simulink library "bushing_forces_lib"  (R2025a)
settings: Solver=VariableStepAuto  StartTime=0.0  StopTime=10.0  RelTol=1e-3
undefined symbols (not defined in the file): b1_radial_max, d_axial, d_axialX, d_axialY, d_axialZ, d_radial, d_tors, d_torsX, d_torsY, d_torsZ, f_axial_dam, f_axial_spr, f_axialX_dam, f_axialX_spr, f_axialY_dam, f_axialY_spr, f_axialZ_dam, f_axialZ_spr, f_radial_dam, f_radial_max, f_radial_spr, k1_radial_max, k_axial, k_axialX, k_axialY, k_axialZ, k_radial, k_tors, k_torsX, k_torsY, k_torsZ, Linear, m, m_spr, m_sprZ, m_torsY, m_torsZ, m_torX, q_spr, q_sprZ, Table, v_axial, v_axialX, v_axialY, v_axialZ, v_radial, w, w_torsY, w_torsZ, w_torX, x_axial, x_axialX, x_axialY, x_axialZ, x_radial, x_radial_max
libraries: nesl_utility x26, fl_lib x18, $bdroot x10
(part 2 of 2)

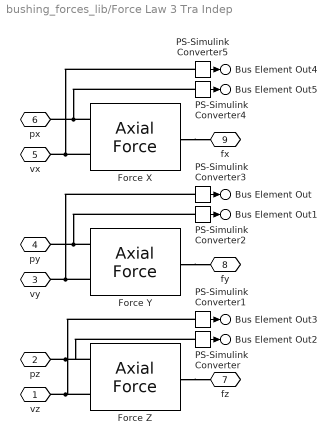
== system bushing_forces_lib/Force Law 3 Tra Indep ==
  Force X : $bdroot/Axial Force  popup_force_law_spr=Linear  k_axial=k_axialX  x_axial=x_axialX  f_axial_spr=f_axialX_spr  popup_force_law_dam=Linear  d_axial=d_axialX  v_axial=v_axialX  f_axial_dam=f_axialX_dam
  Force Y : $bdroot/Axial Force  popup_force_law_spr=Linear  k_axial=k_axialY  x_axial=x_axialY  f_axial_spr=f_axialY_spr  popup_force_law_dam=Linear  d_axial=d_axialY  v_axial=v_axialY  f_axial_dam=f_axialY_dam
  Force Z : $bdroot/Axial Force  popup_force_law_spr=Linear  k_axial=k_axialZ  x_axial=x_axialZ  f_axial_spr=f_axialZ_spr  popup_force_law_dam=Linear  d_axial=d_axialZ  v_axial=v_axialZ  f_axial_dam=f_axialZ_dam
  PS-Simulink Converter : nesl_utility/PS-Simulink Converter  PhysicalDomain=network_engine_domain  SubClassName=ps_output  LeftPortType=input  RightPortType=output  PseudoPeriodic=off  Frequencies=[]  VectorFormat=inherit  Unit=mm  AffineConversion=off
  PS-Simulink Converter1 : nesl_utility/PS-Simulink Converter  PhysicalDomain=network_engine_domain  SubClassName=ps_output  LeftPortType=input  RightPortType=output  PseudoPeriodic=off  Frequencies=[]  VectorFormat=inherit  Unit=m/s  AffineConversion=off
  PS-Simulink Converter2 : nesl_utility/PS-Simulink Converter  PhysicalDomain=network_engine_domain  SubClassName=ps_output  LeftPortType=input  RightPortType=output  PseudoPeriodic=off  Frequencies=[]  VectorFormat=inherit  Unit=mm  AffineConversion=off
  PS-Simulink Converter3 : nesl_utility/PS-Simulink Converter  PhysicalDomain=network_engine_domain  SubClassName=ps_output  LeftPortType=input  RightPortType=output  PseudoPeriodic=off  Frequencies=[]  VectorFormat=inherit  Unit=m/s  AffineConversion=off
  PS-Simulink Converter4 : nesl_utility/PS-Simulink Converter  PhysicalDomain=network_engine_domain  SubClassName=ps_output  LeftPortType=input  RightPortType=output  PseudoPeriodic=off  Frequencies=[]  VectorFormat=inherit  Unit=mm  AffineConversion=off
  PS-Simulink Converter5 : nesl_utility/PS-Simulink Converter  PhysicalDomain=network_engine_domain  SubClassName=ps_output  LeftPortType=input  RightPortType=output  PseudoPeriodic=off  Frequencies=[]  VectorFormat=inherit  Unit=m/s  AffineConversion=off
  vz : PMIOPort  Side=Right
  pz : PMIOPort  Port=2  Side=Right
  vy : PMIOPort  Port=3  Side=Right
  py : PMIOPort  Port=4  Side=Right
  vx : PMIOPort  Port=5  Side=Right
  px : PMIOPort  Port=6  Side=Right
  fz : PMIOPort  Port=7  Side=Left
  fy : PMIOPort  Port=8  Side=Left
  fx : PMIOPort  Port=9  Side=Left
  Bus Element Out : Outport  PortName=m  Element=vy
  Bus Element Out1 : Outport  PortName=m  Element=py
  Bus Element Out2 : Outport  PortName=m  Element=pz
  Bus Element Out3 : Outport  PortName=m  Element=vz
  Bus Element Out4 : Outport  PortName=m  Element=vx
  Bus Element Out5 : Outport  PortName=m  Element=px
  wires:
  PS-Simulink Converter1/1 -> Bus Element Out3/1
  PS-Simulink Converter/1 -> Bus Element Out2/1
  PS-Simulink Converter3/1 -> Bus Element Out/1
  PS-Simulink Converter2/1 -> Bus Element Out1/1
  PS-Simulink Converter4/1 -> Bus Element Out5/1
  PS-Simulink Converter5/1 -> Bus Element Out4/1
  connections:
  vz/RConn1 -- Force Z/LConn2 -- PS-Simulink Converter1/LConn1
  Force Z/RConn1 -- fz/RConn1
  pz/RConn1 -- Force Z/LConn1 -- PS-Simulink Converter/LConn1
  Force Y/RConn1 -- fy/RConn1
  Force X/RConn1 -- fx/RConn1
  PS-Simulink Converter2/LConn1 -- Force Y/LConn1 -- py/RConn1
  PS-Simulink Converter4/LConn1 -- Force X/LConn1 -- px/RConn1
  PS-Simulink Converter5/LConn1 -- Force X/LConn2 -- vx/RConn1
  PS-Simulink Converter3/LConn1 -- Force Y/LConn2 -- vy/RConn1

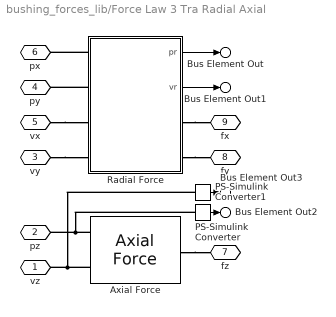
== system bushing_forces_lib/Force Law 3 Tra Radial Axial ==
  Axial Force : $bdroot/Axial Force  popup_force_law_spr=Linear  k_axial=k_axial  x_axial=x_axial  f_axial_spr=f_axial_spr  popup_force_law_dam=Linear  d_axial=d_axial  v_axial=v_axial  f_axial_dam=f_axial_dam
  PS-Simulink Converter : nesl_utility/PS-Simulink Converter  PhysicalDomain=network_engine_domain  SubClassName=ps_output  LeftPortType=input  RightPortType=output  PseudoPeriodic=off  Frequencies=[]  VectorFormat=inherit  Unit=mm  AffineConversion=off
  PS-Simulink Converter1 : nesl_utility/PS-Simulink Converter  PhysicalDomain=network_engine_domain  SubClassName=ps_output  LeftPortType=input  RightPortType=output  PseudoPeriodic=off  Frequencies=[]  VectorFormat=inherit  Unit=m/s  AffineConversion=off
  Radial Force : Subsystem  mask(Radial Compliance){popup_force_law_spr=Linear, k_radial=k_radial, f_radial_spr=f_radial_spr, x_radial=x_radial, k1_radial_max=k1_radial_max, b1_radial_max=b1_radial_max, x_radial_max=x_radial_max, f_radial_max=f_radial_max, popup_force_law_dam=Linear, d_radial=d_radial, v_radial=v_radial, f_radial_dam=f_radial_dam}
      mask prompts: popup_force_law_spr "Spring Force Law"; k_radial "Spring Coefficient (N/mm)"; f_radial_spr "Spring Force [min max] (N)"; x_radial "Spring Deflection [min max] (mm)"; k1_radial_max "Maxwell k1"; b1_radial_max "Maxwell b1"; x_radial_max "Maxwell Displacement [min max] (mm)"; f_radial_max "Maxwell Force [min max] (N)"; popup_force_law_dam "Damper Force Law"; d_radial "Damper Coefficient (N/(m/s))"; v_radial "Damper Velocity [min max] (m/s)"; f_radial_dam "Damper Force [min max] (N)"
      mask help: Models radial compliance of the bushing. Select force laws that model compliance as linear, nonlinear, or nonlinear with hysteresis.
      mask TypeOptions popup_force_law_spr: Force Law Spring/popup_force_law
      mask Callback popup_force_law_spr:
      | maskObj = Simulink.Mask.get(gcb); % Get the mask object of the current block
      | krad_h  = maskObj.getParameter('k_radial'); % Get the parameter to hide
      | 
      | xrad_h  = maskObj.getParameter('x_radial'); % Get the parameter to hide
      | fSrad_h = maskObj.getParameter('f_radial_spr'); % Get the parameter to hide
      | k1rad_h = maskObj.getParameter('k1_radial_max'); % Get the parameter to hide
      | b1rad_h = maskObj.getParameter('b1_radial_max'); % Get the parameter to hide
      | xmrad_h = maskObj.getParameter('x_radial_max'); % Get the parameter to hide
      | fmrad_h = maskObj.getParameter('f_radial_max'); % Get the parameter to hide
      | 
      | % Check the value of ControlParam
      | frcLawSpr = get_param(gcb, 'popup_force_law_spr');
      | 
      | krad_h.Visible  = 'off';
      | xrad_h.Visible  = 'off';
      | fSrad_h.Visible = 'off';
      | k1rad_h.Visible  = 'off';
      | b1rad_h.Visible  = 'off';
      | xmrad_h.Visible  = 'off';
      | fmrad_h.Visible  = 'off';
      | 
      | if strcmp(frcLawSpr, 'Linear')
      |     krad_h.Visible  = 'on';
      | elseif strcmp(frcLawSpr, 'Table')
      |     xrad_h.Visible  = 'on';
      |     fSrad_h.Visible = 'on';
      | elseif strcmp(frcLawSpr, 'Maxwell_SLS')
      |     k1rad_h.Visible  = 'on';
      |     b1rad_h.Visible = 'on';
      |     xmrad_h.Visible = 'on';
      |     fmrad_h.Visible = 'on';
      | end
      mask TypeOptions k_radial: Force Law Spring/k_radial
      mask TypeOptions f_radial_spr: Force Law Spring/f_radial
      mask TypeOptions x_radial: Force Law Spring/x_radial
      mask TypeOptions k1_radial_max: Force Law Spring/k1_radial_max
      mask TypeOptions b1_radial_max: Force Law Spring/b1_radial_max
      mask TypeOptions x_radial_max: Force Law Spring/x_radial_max
      mask TypeOptions f_radial_max: Force Law Spring/f_radial_max
      mask TypeOptions popup_force_law_dam: Force Law Damping/popup_force_law
      mask Callback popup_force_law_dam:
      | maskObj = Simulink.Mask.get(gcb); % Get the mask object of the current block
      | drad_h  = maskObj.getParameter('d_radial'); % Get the parameter to hide
      | 
      | vrad_h  = maskObj.getParameter('v_radial'); % Get the parameter to hide
      | fDrad_h = maskObj.getParameter('f_radial_dam'); % Get the parameter to hide
      | 
      | % Check the value of ControlParam
      | frcLawDam = get_param(gcb, 'popup_force_law_dam');
      | 
      | drad_h.Visible  = 'off';
      | vrad_h.Visible  = 'off';
      | fDrad_h.Visible = 'off';
      | 
      | if strcmp(frcLawDam, 'Linear')
      |     drad_h.Visible  = 'on';
      | elseif strcmp(frcLawDam, 'Table')
      |     vrad_h.Visible  = 'on';
      |     fDrad_h.Visible = 'on';
      | end
      mask TypeOptions d_radial: Force Law Damping/d_radial
      mask TypeOptions v_radial: Force Law Damping/v_radial
      mask TypeOptions f_radial_dam: Force Law Damping/f_radial
      mask DialogControl cont_radial Prompt: Radial
  vz : PMIOPort  Side=Right
  pz : PMIOPort  Port=2  Side=Right
  vy : PMIOPort  Port=3  Side=Right
  py : PMIOPort  Port=4  Side=Right
  vx : PMIOPort  Port=5  Side=Right
  px : PMIOPort  Port=6  Side=Right
  fz : PMIOPort  Port=7  Side=Left
  fy : PMIOPort  Port=8  Side=Left
  fx : PMIOPort  Port=9  Side=Left
  Bus Element Out : Outport  PortName=m  Element=pr
  Bus Element Out1 : Outport  PortName=m  Element=vr
  Bus Element Out2 : Outport  PortName=m  Element=pa
  Bus Element Out3 : Outport  PortName=m  Element=va
  wires:
  Radial Force/2(vr) -> Bus Element Out1/1
  Radial Force/1(pr) -> Bus Element Out/1
  PS-Simulink Converter/1 -> Bus Element Out2/1
  PS-Simulink Converter1/1 -> Bus Element Out3/1
  connections:
  vy/RConn1 -- Radial Force/LConn4
  vx/RConn1 -- Radial Force/LConn3
  Radial Force/LConn1 -- px/RConn1
  Radial Force/LConn2 -- py/RConn1
  Radial Force/RConn1 -- fx/RConn1
  Radial Force/RConn2 -- fy/RConn1
  PS-Simulink Converter/LConn1 -- Axial Force/LConn1 -- pz/RConn1
  Axial Force/RConn1 -- fz/RConn1
  PS-Simulink Converter1/LConn1 -- Axial Force/LConn2 -- vz/RConn1

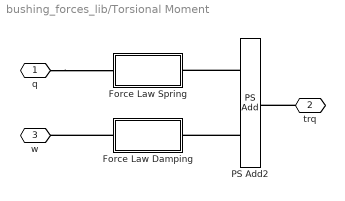
== system bushing_forces_lib/Torsional Moment ==
  Force Law Damping : Subsystem  Variant=on  VariantControlMode=label  VariantControl=Choice  LabelModeActiveChoice=Linear  mask(Compliance Damping){popup_force_law=Linear, d_tors=d_tors, w=w, m=m}
      mask prompts: popup_force_law "Force Law"; d_tors "Linear Damping (N*m/(deg/s))"; w "Table Omega (deg/s)"; m "Table Torque (N*m)"
      mask help: Models damping of the compliance element using linear or nonlinear models.
      mask init:
      | if(strcmp(get_param(gcb, 'popup_force_law'),'Linear'))
      |     set_param(gcb,'LabelModeActiveChoice','Linear')
      | else
      |     set_param(gcb,'LabelModeActiveChoice','Table')
      | end
      mask TypeOptions popup_force_law: Linear | Table
      mask Callback popup_force_law:
      | maskObj = Simulink.Mask.get(gcb); % Get the mask object of the current block
      | dtor_h  = maskObj.getParameter('d_tors'); % Get the parameter to hide
      | 
      | w_h  = maskObj.getParameter('w'); % Get the parameter to hide
      | m_h = maskObj.getParameter('m'); % Get the parameter to hide
      | 
      | % Check the value of ControlParam
      | controlParamValue = get_param(gcb, 'popup_force_law');
      | 
      | dtor_h.Visible  = 'off';
      | w_h.Visible  = 'off';
      | m_h.Visible = 'off';
      | 
      | if strcmp(controlParamValue, 'Linear')
      |     dtor_h.Visible  = 'on';
      | else
      |     w_h.Visible  = 'on';
      |     m_h.Visible = 'on';
      | end
  Force Law Spring : Subsystem  Variant=on  VariantControlMode=label  VariantControl=Choice  LabelModeActiveChoice=Linear  mask(Compliance Stiffness){popup_force_law=Linear, k_tors=k_tors, q=q_spr, m=m_spr}
      mask prompts: popup_force_law "Force Law"; k_tors "Linear Stiffness (N*m/deg)"; q "Table Displacement (deg)"; m "Table Torque (N*m)"
      mask help: Models stiffness of the compliance element using linear or nonlinear models.
      mask init:
      | if(strcmp(get_param(gcb, 'popup_force_law'),'Linear'))
      |     set_param(gcb,'LabelModeActiveChoice','Linear')
      | else
      |     set_param(gcb,'LabelModeActiveChoice','Table')
      | end
      mask TypeOptions popup_force_law: Linear | Table
      mask Callback popup_force_law:
      | maskObj = Simulink.Mask.get(gcb); % Get the mask object of the current block
      | ktor_h  = maskObj.getParameter('k_tors'); % Get the parameter to hide
      | 
      | q_h  = maskObj.getParameter('q'); % Get the parameter to hide
      | m_h  = maskObj.getParameter('m'); % Get the parameter to hide
      | 
      | % Check the value of ControlParam
      | controlParamValue = get_param(gcb, 'popup_force_law');
      | 
      | krad_h.Visible  = 'off';
      | q_h.Visible  = 'off';
      | m_h.Visible  = 'off';
      | 
      | if strcmp(controlParamValue, 'Linear')
      |     krad_h.Visible  = 'on';
      | else
      |     q_h.Visible  = 'on';
      |     m_h.Visible  = 'on';
      | end
  PS Add2 : fl_lib/Physical Signals/Functions/PS Add
  q : PMIOPort  Side=Left
  trq : PMIOPort  Port=2  Side=Right
  w : PMIOPort  Port=3  Side=Left
  connections:
  PS Add2/LConn1 -- Force Law Spring/RConn1
  q/RConn1 -- Force Law Spring/LConn1
  Force Law Damping/LConn1 -- w/RConn1
  PS Add2/LConn2 -- Force Law Damping/RConn1
  trq/RConn1 -- PS Add2/RConn1

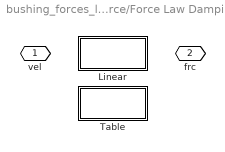
== system bushing_forces_lib/Axial Force/Force Law Damping ==
  Linear : Subsystem  VariantControl=Linear  mask(Linear Damping){b=d_axial}
      mask prompts: b "Damping (N/(m/s))"
      mask help: Models linear damping.
      mask TypeOptions b: Damping/gain
  Table : Subsystem  VariantControl=Table  mask(Nonlinear Damping){x=v_axial, f=f_axial}
      mask prompts: x "Speed (m/s)"; f "Force (N)"
      mask help: Models nonlinear damping using a lookup table.
      mask TypeOptions x: PS Lookup Table (1D)/x
      mask TypeOptions f: PS Lookup Table (1D)/f
  vel : PMIOPort  Side=Left
  frc : PMIOPort  Port=2  Side=Right

== system bushing_forces_lib/Axial Force/Force Law Spring ==
  Linear : Subsystem  VariantControl=Linear  mask(Linear Stiffness){k=k_axial}
      mask prompts: k "Stiffness (N/mm)"
      mask help: Models linear stiffness.
      mask TypeOptions k: Stiffness/gain
  Table : Subsystem  VariantControl=Table  mask(Nonlinear Stiffness){x=x_axial, f=f_axial}
      mask prompts: x "Displacement (mm)"; f "Force (N)"
      mask help: Models nonlinear stiffness using a lookup table.
      mask TypeOptions x: PS Lookup Table (1D)/x
      mask TypeOptions f: PS Lookup Table (1D)/f
  def : PMIOPort  Side=Left
  frc : PMIOPort  Port=2  Side=Right

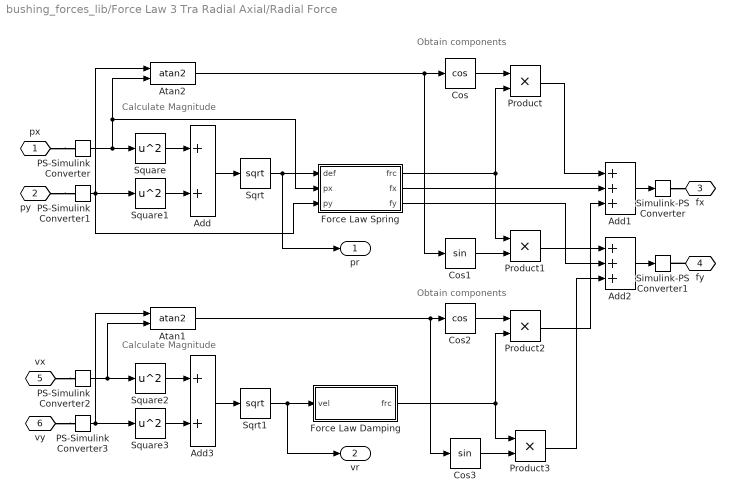
== system bushing_forces_lib/Force Law 3 Tra Radial Axial/Radial Force ==
  note: Obtain components
  note: Calculate Magnitude
  note: Obtain components
  note: Calculate Magnitude
  Add : Sum
  Add1 : Sum  Inputs=+++
  Add2 : Sum  Inputs=+++
  Add3 : Sum
  Atan1 : Trigonometry  Operator=atan2
  Atan2 : Trigonometry  Operator=atan2
  Cos : Trigonometry  Operator=cos
  Cos1 : Trigonometry
  Cos2 : Trigonometry  Operator=cos
  Cos3 : Trigonometry
  Force Law Damping : Subsystem  Variant=on  VariantControlMode=label  VariantControl=Choice  LabelModeActiveChoice=Linear  mask(Compliance Damping){popup_force_law=Linear, d_radial=d_radial, v_radial=v_radial, f_radial=f_radial_dam}
      mask prompts: popup_force_law "Damper Force Law"; d_radial "Damper Coefficient (N/(m/s))"; v_radial "Damper Velocity (m/s)"; f_radial "Damper Force (N)"
      mask help: Models damping of the compliance element using linear or nonlinear models.
      mask init:
      | fLawChoice = get_param(gcb, 'popup_force_law');
      | set_param(gcb,'LabelModeActiveChoice',fLawChoice);
      mask TypeOptions popup_force_law: Linear | Table
      mask Callback popup_force_law:
      | maskObj = Simulink.Mask.get(gcb); % Get the mask object of the current block
      | drad_h  = maskObj.getParameter('d_radial'); % Get the parameter to hide
      | 
      | vrad_h  = maskObj.getParameter('v_radial'); % Get the parameter to hide
      | frad_h = maskObj.getParameter('f_radial'); % Get the parameter to hide
      | 
      | % Check the value of ControlParam
      | controlParamValue = get_param(gcb, 'popup_force_law');
      | 
      | drad_h.Visible  = 'off';
      | vrad_h.Visible  = 'off';
      | frad_h.Visible = 'off';
      | 
      | if strcmp(controlParamValue, 'Linear')
      |     drad_h.Visible  = 'on';
      | elseif strcmp(controlParamValue, 'Table')
      |     vrad_h.Visible = 'on';
      |     frad_h.Visible = 'on';
      | end
  Force Law Spring : Subsystem  Variant=on  VariantControlMode=label  VariantControl=Choice  LabelModeActiveChoice=Linear  mask(Compliance Stiffness){popup_force_law=Linear, k_radial=k_radial, x_radial=x_radial, f_radial=f_radial_spr, k1_radial_max=k1_radial_max, b1_radial_max=b1_radial_max, x_radial_max=x_radial_max, f_radial_max=f_radial_max}
      mask prompts: popup_force_law "Spring Force Law"; k_radial "Spring Coefficient (N/mm)"; x_radial "Spring Displacement [min max] (mm)"; f_radial "Spring Force [min max] (N)"; k1_radial_max "Maxwell k1"; b1_radial_max "Maxwell b1"; x_radial_max "Maxwell Displacement [min max] (mm)"; f_radial_max "Maxwell Force [min max] (N)"
      mask help: Models stiffness of the compliance element using linear, nonlinear, or nonlinear with hysteresis models.
      mask init:
      | fLawChoice = get_param(gcb, 'popup_force_law');
      | set_param(gcb,'LabelModeActiveChoice',fLawChoice);
      mask TypeOptions popup_force_law: Linear | Table | Maxwell_SLS
      mask Callback popup_force_law:
      | maskObj = Simulink.Mask.get(gcb); % Get the mask object of the current block
      | krad_h  = maskObj.getParameter('k_radial'); % Get the parameter to hide
      | 
      | xrad_h  = maskObj.getParameter('x_radial'); % Get the parameter to hide
      | frad_h  = maskObj.getParameter('f_radial'); % Get the parameter to hide
      | k1rad_h = maskObj.getParameter('k1_radial_max'); % Get the parameter to hide
      | b1rad_h = maskObj.getParameter('b1_radial_max'); % Get the parameter to hide
      | xmrad_h = maskObj.getParameter('x_radial_max'); % Get the parameter to hide
      | fmrad_h = maskObj.getParameter('f_radial_max'); % Get the parameter to hide
      | 
      | 
      | % Check the value of ControlParam
      | controlParamValue = get_param(gcb, 'popup_force_law');
      | 
      | krad_h.Visible  = 'off';
      | xrad_h.Visible  = 'off';
      | frad_h.Visible  = 'off';
      | k1rad_h.Visible  = 'off';
      | b1rad_h.Visible  = 'off';
      | xmrad_h.Visible  = 'off';
      | fmrad_h.Visible  = 'off';
      | 
      | if strcmp(controlParamValue, 'Linear')
      |     krad_h.Visible  = 'on';
      | elseif strcmp(controlParamValue, 'Table')
      |     xrad_h.Visible  = 'on';
      |     frad_h.Visible = 'on';
      | elseif strcmp(controlParamValue, 'Maxwell_SLS')
      |     k1rad_h.Visible  = 'on';
      |     b1rad_h.Visible = 'on';
      |     xmrad_h.Visible = 'on';
      |     fmrad_h.Visible = 'on';
      | end
  PS-Simulink Converter : nesl_utility/PS-Simulink Converter  PhysicalDomain=network_engine_domain  SubClassName=ps_output  LeftPortType=input  RightPortType=output  PseudoPeriodic=off  Frequencies=[]  VectorFormat=inherit  Unit=mm  AffineConversion=off
  PS-Simulink Converter1 : nesl_utility/PS-Simulink Converter  PhysicalDomain=network_engine_domain  SubClassName=ps_output  LeftPortType=input  RightPortType=output  PseudoPeriodic=off  Frequencies=[]  VectorFormat=inherit  Unit=mm  AffineConversion=off
  PS-Simulink Converter2 : nesl_utility/PS-Simulink Converter  PhysicalDomain=network_engine_domain  SubClassName=ps_output  LeftPortType=input  RightPortType=output  PseudoPeriodic=off  Frequencies=[]  VectorFormat=inherit  Unit=m/s  AffineConversion=off
  PS-Simulink Converter3 : nesl_utility/PS-Simulink Converter  PhysicalDomain=network_engine_domain  SubClassName=ps_output  LeftPortType=input  RightPortType=output  PseudoPeriodic=off  Frequencies=[]  VectorFormat=inherit  Unit=m/s  AffineConversion=off
  Product{,1..3} (4 alike) : Product
  Simulink-PS Converter : nesl_utility/Simulink-PS Converter  PhysicalDomain=network_engine_domain  SubClassName=ps_input  LeftPortType=input  RightPortType=output  PseudoPeriodic=off  Frequencies=[]  NoiseDistribution=none  NoiseParameters=[]  Unit=1  AffineConversion=off  FilteringAndDerivatives=provide  SimscapeFilterOrder=1  InputFilterTimeConstant=0.001  UdotUserProvided=0
  Simulink-PS Converter1 : nesl_utility/Simulink-PS Converter  PhysicalDomain=network_engine_domain  SubClassName=ps_input  LeftPortType=input  RightPortType=output  PseudoPeriodic=off  Frequencies=[]  NoiseDistribution=none  NoiseParameters=[]  Unit=1  AffineConversion=off  FilteringAndDerivatives=provide  SimscapeFilterOrder=1  InputFilterTimeConstant=0.001  UdotUserProvided=0
  Sqrt : Sqrt
  Sqrt1 : Sqrt
  Square{,1..3} (4 alike) : Math  Operator=square
  px : PMIOPort  Side=Left
  py : PMIOPort  Port=2  Side=Left
  fx : PMIOPort  Port=3  Side=Right
  fy : PMIOPort  Port=4  Side=Right
  vx : PMIOPort  Port=5  Side=Left
  vy : PMIOPort  Port=6  Side=Left
  pr : Outport
  vr : Outport  Port=2
  wires:
  Add2/1 -> Simulink-PS Converter1/1
  Product3/1 -> Add2/3
  Product2/1 -> Add1/3
  Force Law Damping/1(frc) -> Product2/2, Product3/1
  Atan1/1 -> Cos2/1, Cos3/1
  Cos2/1 -> Product2/1
  Cos3/1 -> Product3/2
  Sqrt1/1 -> Force Law Damping/1(vel), vr/1
  PS-Simulink Converter2/1 -> Atan1/2, Square2/1
  PS-Simulink Converter3/1 -> Atan1/1, Square3/1
  Square2/1 -> Add3/1
  Square3/1 -> Add3/2
  Add3/1 -> Sqrt1/1
  Force Law Spring/3(fy) -> Add2/2
  Product1/1 -> Add2/1
  Cos1/1 -> Product1/2
  Add1/1 -> Simulink-PS Converter/1
  Force Law Spring/2(fx) -> Add1/2
  Product/1 -> Add1/1
  Force Law Spring/1(frc) -> Product/2, Product1/1
  Cos/1 -> Product/1
  Atan2/1 -> Cos1/1, Cos/1
  Sqrt/1 -> Force Law Spring/1(def), pr/1
  Add/1 -> Sqrt/1
  Square1/1 -> Add/2
  Square/1 -> Add/1
  PS-Simulink Converter1/1 -> Square1/1, Atan2/1, Force Law Spring/3(py)
  PS-Simulink Converter/1 -> Square/1, Force Law Spring/2(px), Atan2/2
  connections:
  fy/RConn1 -- Simulink-PS Converter1/RConn1
  Simulink-PS Converter/RConn1 -- fx/RConn1
  vy/RConn1 -- PS-Simulink Converter3/LConn1
  vx/RConn1 -- PS-Simulink Converter2/LConn1
  py/RConn1 -- PS-Simulink Converter1/LConn1
  px/RConn1 -- PS-Simulink Converter/LConn1

== system bushing_forces_lib/Torsional Moment/Force Law Damping ==
  Linear : Subsystem  VariantControl=Linear  mask(Linear Damping){d_tors=d_tors}
      mask prompts: d_tors "Damping (N*m/(deg/s))"
      mask help: Models linear damping.
      mask TypeOptions d_tors: Damping/gain
  Table : Subsystem  VariantControl=Table  mask(Nonlinear Damping){w=w, m=m}
      mask prompts: w "Table grid vector"; m "Table values"
      mask help: Models nonlinear damping using a lookup table.
      mask TypeOptions w: PS Lookup Table (1D)/x
      mask TypeOptions m: PS Lookup Table (1D)/f
  vel : PMIOPort  Side=Left
  trq : PMIOPort  Port=2  Side=Right

== system bushing_forces_lib/Torsional Moment/Force Law Spring ==
  Linear : Subsystem  VariantControl=Linear  mask(Linear Stiffness){k_tors=k_tors}
      mask prompts: k_tors "Stiffness (N*m/deg)"
      mask help: Models linear stiffness.
      mask TypeOptions k_tors: Stiffness/gain
  Table : Subsystem  VariantControl=Table  mask(Nonlinear Stiffness){q=q, m=m}
      mask prompts: q "Displacement (deg)"; m "Torque (N*m)"
      mask help: Models nonlinear stiffness using a lookup table.
      mask TypeOptions q: PS Lookup Table (1D)/x
      mask TypeOptions m: PS Lookup Table (1D)/f
  def : PMIOPort  Side=Left
  frc : PMIOPort  Port=2  Side=Right

== system bushing_forces_lib/Axial Force/Force Law Damping/Linear ==
  Attract : fl_lib/Physical Signals/Functions/PS Gain  gain=-1
  Damping : fl_lib/Physical Signals/Functions/PS Gain  gain=b N/(m/s)
  vel : PMIOPort  Side=Left
  frc : PMIOPort  Port=2  Side=Right
  connections:
  Attract/RConn1 -- frc/RConn1
  Damping/LConn1 -- vel/RConn1
  Damping/RConn1 -- Attract/LConn1

== system bushing_forces_lib/Axial Force/Force Law Damping/Table ==
  Attract : fl_lib/Physical Signals/Functions/PS Gain  gain=-1
  PS Lookup Table (1D) : fl_lib/Physical Signals/Lookup Tables/PS Lookup Table (1D)  x=x m/s  f=f N  interp_method=simscape.enum.interpolation.linear  extrap_method=simscape.enum.extrapolation.linear
  vel : PMIOPort  Side=Left
  frc : PMIOPort  Port=2  Side=Right
  connections:
  PS Lookup Table (1D)/RConn1 -- Attract/LConn1
  PS Lookup Table (1D)/LConn1 -- vel/RConn1
  Attract/RConn1 -- frc/RConn1

== system bushing_forces_lib/Axial Force/Force Law Spring/Linear ==
  Attract : fl_lib/Physical Signals/Functions/PS Gain  gain=-1
  Stiffness : fl_lib/Physical Signals/Functions/PS Gain  gain=k N/mm
  def : PMIOPort  Side=Left
  frc : PMIOPort  Port=2  Side=Right
  connections:
  Stiffness/RConn1 -- Attract/LConn1
  Stiffness/LConn1 -- def/RConn1
  Attract/RConn1 -- frc/RConn1

== system bushing_forces_lib/Axial Force/Force Law Spring/Table ==
  Attract : fl_lib/Physical Signals/Functions/PS Gain  gain=-1
  PS Lookup Table (1D) : fl_lib/Physical Signals/Lookup Tables/PS Lookup Table (1D)  x=x mm  f=f N  interp_method=simscape.enum.interpolation.linear  extrap_method=simscape.enum.extrapolation.linear
  def : PMIOPort  Side=Left
  frc : PMIOPort  Port=2  Side=Right
  connections:
  Attract/RConn1 -- frc/RConn1
  PS Lookup Table (1D)/LConn1 -- def/RConn1
  PS Lookup Table (1D)/RConn1 -- Attract/LConn1

== system bushing_forces_lib/Force Law 3 Tra Radial Axial/Radial Force/Force Law Damping ==
  vel : Inport
  Linear : Subsystem  VariantControl=Linear  mask(Linear Damping){b=d_radial}
      mask prompts: b "Damping (N/(m/s))"
      mask help: Models linear damping.
      mask TypeOptions b: Damping/gain
  Table : Subsystem  VariantControl=Table  mask(Nonlinear Damping){x=v_radial, f=f_radial}
      mask prompts: x "Speed (m/s)"; f "Force (N)"
      mask help: Models nonlinear damping using a lookup table.
  frc : Outport

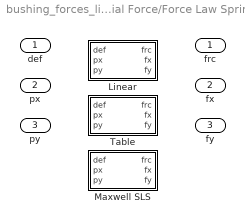
== system bushing_forces_lib/Force Law 3 Tra Radial Axial/Radial Force/Force Law Spring ==
  def : Inport
  px : Inport  Port=2
  py : Inport  Port=3
  Linear : Subsystem  VariantControl=Linear  mask(Linear stiffness){k=k_radial}
      mask prompts: k "Stiffness (N/mm)"
      mask help: Models linear stiffness.
      mask TypeOptions k: Stiffness/gain
  Maxwell SLS : Subsystem  VariantControl=Maxwell_SLS  mask(Nonlinear Stiffness with Hysteresis){k1_maxwell=k1_radial_max, b1_maxwell=b1_radial_max, x=x_radial_max, f=f_radial_max}
      mask prompts: k1_maxwell "Coefficient k1"; b1_maxwell "Coefficient b1"; x "Spring Deflection [min max] (mm)"; f "Spring Force [min max] (N)"
      mask help: Models nonlinear stiffness with hysteresis. This model is similar to the Maxwell SLS model with a series spring-damper in parallel with a nonlinear spring. The coefficients are used in a transfer function to model the series spring damper. (k1*b1s)/(b1*s + k1)
  Table : Subsystem  VariantControl=Table  mask(Nonlinear Stiffness){x=x_radial, f=f_radial}
      mask prompts: x "Displacement (mm)"; f "Force (N)"
      mask help: Models nonlinear stiffness using a lookup table.
  frc : Outport
  fx : Outport  Port=2
  fy : Outport  Port=3

== system bushing_forces_lib/Torsional Moment/Force Law Damping/Linear ==
  Attract : fl_lib/Physical Signals/Functions/PS Gain  gain=-1
  Damping : fl_lib/Physical Signals/Functions/PS Gain  gain=d_tors N*m/(deg/s)
  vel : PMIOPort  Side=Left
  trq : PMIOPort  Port=2  Side=Right
  connections:
  Damping/RConn1 -- Attract/LConn1
  Damping/LConn1 -- vel/RConn1
  Attract/RConn1 -- trq/RConn1

== system bushing_forces_lib/Torsional Moment/Force Law Damping/Table ==
  Attract : fl_lib/Physical Signals/Functions/PS Gain  gain=-1
  PS Lookup Table (1D) : fl_lib/Physical Signals/Lookup Tables/PS Lookup Table (1D)  x=w deg/s  f=m N*m  interp_method=simscape.enum.interpolation.linear  extrap_method=simscape.enum.extrapolation.linear
  vel : PMIOPort  Side=Left
  trq : PMIOPort  Port=2  Side=Right
  connections:
  Attract/RConn1 -- trq/RConn1
  PS Lookup Table (1D)/LConn1 -- vel/RConn1
  PS Lookup Table (1D)/RConn1 -- Attract/LConn1

== system bushing_forces_lib/Torsional Moment/Force Law Spring/Linear ==
  Attract : fl_lib/Physical Signals/Functions/PS Gain  gain=-1
  Stiffness : fl_lib/Physical Signals/Functions/PS Gain  gain=k_tors N*m/deg
  def : PMIOPort  Side=Left
  frc : PMIOPort  Port=2  Side=Right
  connections:
  Attract/RConn1 -- frc/RConn1
  Stiffness/LConn1 -- def/RConn1
  Stiffness/RConn1 -- Attract/LConn1

== system bushing_forces_lib/Torsional Moment/Force Law Spring/Table ==
  Attract : fl_lib/Physical Signals/Functions/PS Gain  gain=-1
  PS Lookup Table (1D) : fl_lib/Physical Signals/Lookup Tables/PS Lookup Table (1D)  x=q deg  f=m N*m  interp_method=simscape.enum.interpolation.linear  extrap_method=simscape.enum.extrapolation.linear
  def : PMIOPort  Side=Left
  frc : PMIOPort  Port=2  Side=Right
  connections:
  PS Lookup Table (1D)/RConn1 -- Attract/LConn1
  PS Lookup Table (1D)/LConn1 -- def/RConn1
  Attract/RConn1 -- frc/RConn1

== system bushing_forces_lib/Force Law 3 Tra Radial Axial/Radial Force/Force Law Damping/Linear ==
  vel : Inport
  Attract : Gain  Gain=-1
  Damping : Gain  Gain=b
  frc : Outport
  wires:
  Attract/1 -> frc/1
  Damping/1 -> Attract/1
  vel/1 -> Damping/1

== system bushing_forces_lib/Force Law 3 Tra Radial Axial/Radial Force/Force Law Damping/Table ==
  vel : Inport
  1-D Lookup Table : Lookup_n-D  NumberOfTableDimensions=1  BreakpointsForDimension1=x  Table=f  InternalRulePriority=Speed  RndMeth=Simplest
  Attract : Gain  Gain=-1
  frc : Outport
  wires:
  Attract/1 -> frc/1
  vel/1 -> 1-D Lookup Table/1
  1-D Lookup Table/1 -> Attract/1

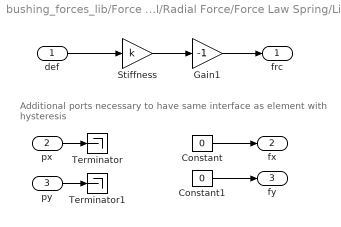
== system bushing_forces_lib/Force Law 3 Tra Radial Axial/Radial Force/Force Law Spring/Linear ==
  note: Additional ports necessary to have same
      |  interface as element with hysteresis
  def : Inport
  px : Inport  Port=2
  py : Inport  Port=3
  Constant : Constant  Value=0
  Constant1 : Constant  Value=0
  Gain1 : Gain  Gain=-1
  Stiffness : Gain  Gain=k
  Terminator : Terminator
  Terminator1 : Terminator
  frc : Outport
  fx : Outport  Port=2
  fy : Outport  Port=3
  wires:
  Constant/1 -> fx/1
  Constant1/1 -> fy/1
  py/1 -> Terminator1/1
  px/1 -> Terminator/1
  Gain1/1 -> frc/1
  Stiffness/1 -> Gain1/1
  def/1 -> Stiffness/1

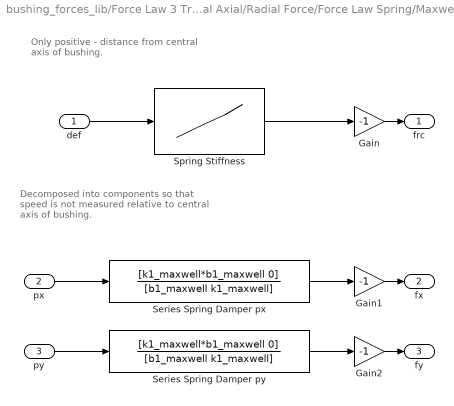
== system bushing_forces_lib/Force Law 3 Tra Radial Axial/Radial Force/Force Law Spring/Maxwell SLS ==
  note: Decomposed into components so that speed is not measured relative to central axis of bushing.
  note: Only positive - distance from central axis of bushing.
  def : Inport
  px : Inport  Port=2
  py : Inport  Port=3
  Gain : Gain  Gain=-1
  Gain1 : Gain  Gain=-1
  Gain2 : Gain  Gain=-1
  Series Spring Damper px : TransferFcn  Numerator=[k1_maxwell*b1_maxwell 0]  Denominator=[b1_maxwell k1_maxwell]
  Series Spring Damper py : TransferFcn  Numerator=[k1_maxwell*b1_maxwell 0]  Denominator=[b1_maxwell k1_maxwell]
  Spring Stiffness : Lookup_n-D  NumberOfTableDimensions=1  BreakpointsForDimension1=x  Table=f  InternalRulePriority=Speed  RndMeth=Simplest
  frc : Outport
  fx : Outport  Port=2
  fy : Outport  Port=3
  wires:
  Gain2/1 -> fy/1
  Gain1/1 -> fx/1
  Series Spring Damper py/1 -> Gain2/1
  Series Spring Damper px/1 -> Gain1/1
  py/1 -> Series Spring Damper py/1
  px/1 -> Series Spring Damper px/1
  def/1 -> Spring Stiffness/1
  Spring Stiffness/1 -> Gain/1
  Gain/1 -> frc/1

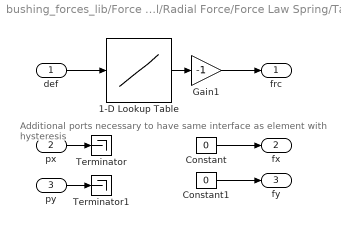
== system bushing_forces_lib/Force Law 3 Tra Radial Axial/Radial Force/Force Law Spring/Table ==
  note: Additional ports necessary to have same
      |  interface as element with hysteresis
  def : Inport
  px : Inport  Port=2
  py : Inport  Port=3
  1-D Lookup Table : Lookup_n-D  NumberOfTableDimensions=1  BreakpointsForDimension1=x  Table=f  InternalRulePriority=Speed  RndMeth=Simplest
  Constant : Constant  Value=0
  Constant1 : Constant  Value=0
  Gain1 : Gain  Gain=-1
  Terminator : Terminator
  Terminator1 : Terminator
  frc : Outport
  fx : Outport  Port=2
  fy : Outport  Port=3
  wires:
  py/1 -> Terminator1/1
  Gain1/1 -> frc/1
  def/1 -> 1-D Lookup Table/1
  Constant1/1 -> fy/1
  Constant/1 -> fx/1
  px/1 -> Terminator/1
  1-D Lookup Table/1 -> Gain1/1
